simulink model "copy_inversed1"  (R2023b)
settings: Solver=VariableStepAuto  StartTime=0.0  StopTime=100  RelTol=1e-3
libraries: simulink_extras x2, slpidlib x1
settings Model: Creator=macbook  LastModifiedBy=user

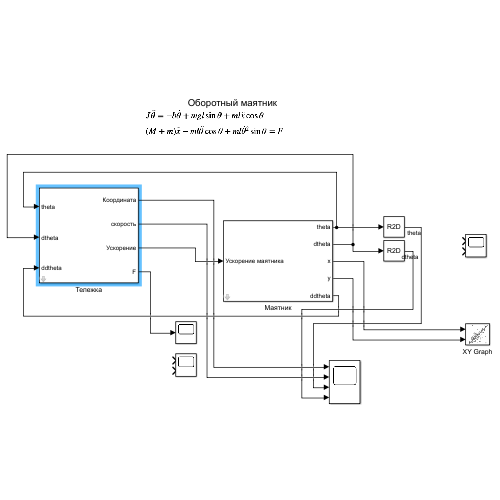
[thumbnail: Simulink's stored preview of the top-level diagram]
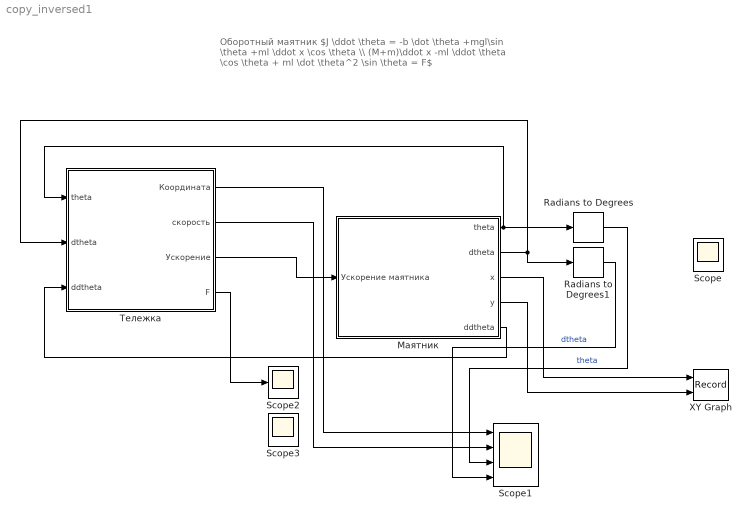
== system copy_inversed1 ==
  note: Оборотный маятник
      | $J \ddot \theta = -b \dot \theta +mgl\sin \theta +ml \ddot x \cos \theta \\ (M+m)\ddot x -ml \ddot \theta \cos \theta + ml \dot \theta^2 \sin \theta = F$
  Radians to Degrees : simulink_extras/Transformations/Radians to Degrees
  Radians to Degrees1 : simulink_extras/Transformations/Radians to Degrees
  Scope : Scope  NumInputPorts=2
  Scope1 : Scope  NumInputPorts=4
  Scope2 : Scope
  Scope3 : Scope  NumInputPorts=2
  XY Graph : Record  FileSettingsInternal="{\"entries\":[{\"content\":{\"excelSettings\":{\"content\":{},\"type\":\"Streamout.ExcelSettings\"}},\"type\":\"Streamout.FileSettingStorage\",\"uuid\":\"\"}],\"packageUris\":[\"http:\\/\\/schema.mathworks.com\\/mf0\\/streamout_blocks\\/R2020a\"],\"version\":\"1.0\"}"  Layout=[1 1]  SignalsInternal="{\"entries\":[{\"content\":{\"signals\":[{\"content\":{\"blockPath\":[],\"dimensions\":[1],\"domain\":\"\",\"lineColor\":\"#a2142f\",\"plots\":[1],\"port\":1,\"sid\":[\"\"],\"signalID\":125,\"signalName\":\"Маятник:3\"},\"type\":\"RecordBlkView.Signal\",\"uuid\":\"\"},{\"content\":{\"blockPath\":[],\"dimensions\":[1],\"domain\":\"\",\"lineColor\":\"#139fff\",\"plots\":[1],\"port\":2,\"sid\":[\"\"],\"signalID\":129,\"signalName\":\"Маятник:4\"},\"type\":\"RecordBlkView.Signal\",\"uuid\":\"\"}]},\"type\":\"RecordBlkView.InputSignals\",\"uuid\":\"\"}],\"packageUris\":[\"http:\\/\\/schema.mathworks.com\\/mf0\\/streamout_blocks\\/R2020a\"],\"version\":\"1.0\"}"  VisualizationBindings="{\"xyplotplugin\":{\"info\":[{\"series\":[{\"bindingParametersList\":[{\"parameter\":\"X-Axis\",\"signalID\":125,\"signalName\":\"Маятник:3\"},{\"parameter\":\"Y-Axis\",\"signalID\":129,\"signalName\":\"Маятник:4\"}],\"seriesID\":60754}],\"subplotID\":1}]}}"  CompatibilityTag=XY
  Маятник : Subsystem  mask{m=0.1, l=0.5, g=9.8, angel=20, b=0.05}
      mask prompts: angel "Начальный угол"
  Тележка : Subsystem  mask{F=0, Mas=1, m=0.1, l=0.5}
      mask prompts: F "начальная F"; Mas "M"
  wires:
  Маятник/1(theta) -> Тележка/1(theta), Radians to Degrees/1
  Radians to Degrees/1 -> Scope1/3  "theta"
  Маятник/3(x) -> XY Graph/1
  Маятник/2(dtheta) -> Тележка/2(dtheta), Radians to Degrees1/1
  Radians to Degrees1/1 -> Scope1/4  "dtheta"
  Маятник/4(y) -> XY Graph/2
  Тележка/4(F) -> Scope2/1
  Тележка/3(Ускорение) -> Маятник/1(Ускорение маятника)
  Маятник/5(ddtheta) -> Тележка/3(ddtheta)
  Тележка/1(Координата) -> Scope1/1
  Тележка/2(скорость) -> Scope1/2

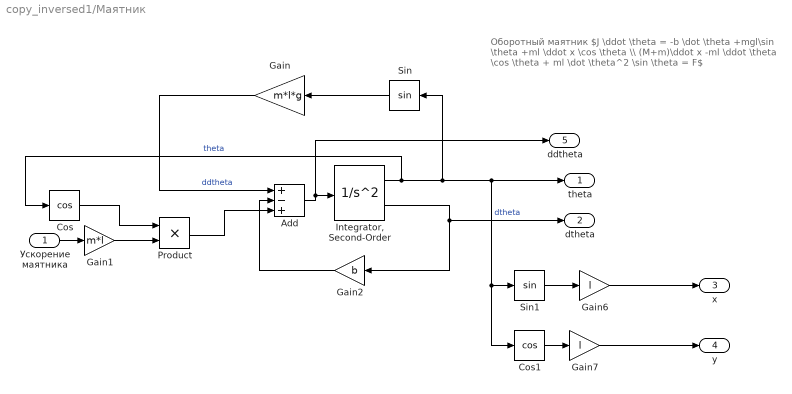
== system copy_inversed1/Маятник ==
  note: Оборотный маятник
      | $J \ddot \theta = -b \dot \theta +mgl\sin \theta +ml \ddot x \cos \theta \\ (M+m)\ddot x -ml \ddot \theta \cos \theta + ml \dot \theta^2 \sin \theta = F$
  Ускорение маятника : Inport
  Add : Sum  Inputs=+-+
  Cos : Trigonometry  Operator=cos
  Cos1 : Trigonometry  Operator=cos
  Gain : Gain  Gain=m*l*g
  Gain1 : Gain  Gain=m*l
  Gain2 : Gain  Gain=b
  Gain6 : Gain  Gain=l
  Gain7 : Gain  Gain=l
  "Integrator, Second-Order" : SecondOrderIntegrator  ICX=deg2rad(angel)  ICDXDT=0
  Product : Product
  Sin : Trigonometry
  Sin1 : Trigonometry
  theta : Outport
  dtheta : Outport  Port=2
  x : Outport  Port=3
  y : Outport  Port=4
  ddtheta : Outport  Port=5
  wires:
  Gain/1 -> Add/1  "ddtheta"
  Add/1 -> ddtheta/1, "Integrator, Second-Order"/1
  Sin1/1 -> Gain6/1
  Gain7/1 -> y/1
  Cos1/1 -> Gain7/1
  "Integrator, Second-Order"/2 -> Gain2/1, dtheta/1  "dtheta"
  "Integrator, Second-Order"/1 -> theta/1, Cos1/1, Sin1/1, Sin/1, Cos/1  "theta"
  Gain2/1 -> Add/2
  Gain6/1 -> x/1
  Sin/1 -> Gain/1
  Ускорение маятника/1 -> Gain1/1
  Gain1/1 -> Product/2
  Cos/1 -> Product/1
  Product/1 -> Add/3

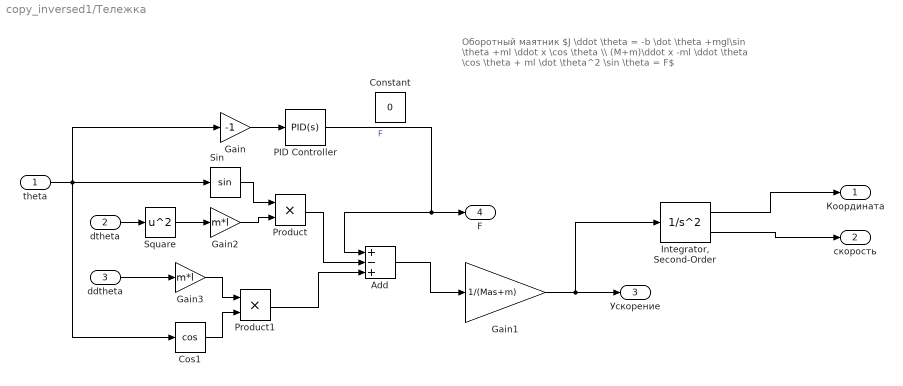
== system copy_inversed1/Тележка ==
  note: Оборотный маятник
      | $J \ddot \theta = -b \dot \theta +mgl\sin \theta +ml \ddot x \cos \theta \\ (M+m)\ddot x -ml \ddot \theta \cos \theta + ml \dot \theta^2 \sin \theta = F$
  theta : Inport
  dtheta : Inport  Port=2
  ddtheta : Inport  Port=3
  Add : Sum  Inputs=+-+
  Constant : Constant  Value=0
  Cos1 : Trigonometry  Operator=cos
  Gain : Gain  Gain=-1
  Gain1 : Gain  Gain=1/(Mas+m)
  Gain2 : Gain  Gain=m*l
  Gain3 : Gain  Gain=m*l
  "Integrator, Second-Order" : SecondOrderIntegrator
  PID Controller : slpidlib/PID Controller  Controller=PID  Form=Parallel  TimeDomain=Continuous-time  UseExternalTs=off  SampleTime=-1  IntegratorMethod=Forward Euler  FilterMethod=Forward Euler  ControllerParametersSource=internal  P=50  I=1  UseKiTs=on  D=50  N=100  UseFilter=on  TunerSelectOption=Transfer Function Based (PID Tuner App)  InitialConditionSource=internal  InitialConditionForIntegrator=0  InitialConditionForFilter=0  DifferentiatorICPrevScaledInput=0  ExternalReset=none  TrackingMode=off  Kt=1  LimitOutput=off  SatLimitsSource=internal  UpperSaturationLimit=inf  LowerSaturationLimit=-inf  LinearizeAsGain=on  AntiWindupMode=none  Kb=1  LimitIntegrator=off  UpperIntegratorSaturationLimit=inf  LowerIntegratorSaturationLimit=-inf  POutMin=[]  POutMax=[]  IOutMin=[]  IOutMax=[]  DOutMin=[]  DOutMax=[]  NOutMin=[]  NOutMax=[]  SumOutMin=[]  SumOutMax=[]  SaturationOutMin=[]  SaturationOutMax=[]  PParamMin=[]  PParamMax=[]  IParamMin=[]  IParamMax=[]  DParamMin=[]  DParamMax=[]  NParamMin=[]  NParamMax=[]  KbParamMin=[]  KbParamMax=[]  KtParamMin=[]  KtParamMax=[]  KbOutMin=[]  KbOutMax=[]  KtOutMin=[]  KtOutMax=[]  IntegratorOutMin=[]  IntegratorOutMax=[]  FilterOutMin=[]  FilterOutMax=[]  SumI1OutMin=[]  SumI1OutMax=[]  SumI2OutMin=[]  SumI2OutMax=[]  SumI3OutMin=[]  SumI3OutMax=[]  SumI4OutMin=[]  SumI4OutMax=[]  SumDOutMin=[]  SumDOutMax=[]  DifferentiatorOutMin=[]  DifferentiatorOutMax=[]  FilterDiffOutCoefMin=[]  FilterDiffOutCoefMax=[]  ReciprocalOutMin=[]  ReciprocalOutMax=[]  SumDenOutMin=[]  SumDenOutMax=[]  SumNumOutMin=[]  SumNumOutMax=[]  DivideOutMin=[]  DivideOutMax=[]  UdiffTsProdOutMin=[]  UdiffTsProdOutMax=[]  NTsProdOutMin=[]  NTsProdOutMax=[]  UintegralTsProdOutMin=[]  UintegralTsProdOutMax=[]  UngainTsProdOutMin=[]  UngainTsProdOutMax=[]  ClampingZeroOutDataTypeStr=Inherit: Inherit via back propagation  ClampingZeroOutMin=[]  ClampingZeroOutMax=[]  FilterDenConstantOutDataTypeStr=Inherit: Inherit via back propagation  FilterDenConstantOutMin=[]  FilterDenConstantOutMax=[]  PCopyOutDataTypeStr=Inherit: Inherit via back propagation  PCopyOutMin=[]  PCopyOutMax=[]  NCopyOutDataTypeStr=Inherit: Inherit via back propagation  NCopyOutMin=[]  NCopyOutMax=[]  IntegratorContinuousStateAttributes=''  IntegratorStateMustResolveToSignalObject=off  IntegratorRTWStateStorageClass=Auto  FilterContinuousStateAttributes=''  FilterStateMustResolveToSignalObject=off  FilterRTWStateStorageClass=Auto  ParallelPVariant=InternalParameters  IdealPVariant=Disabled  IVariant=InternalParameters  DVariant=InternalParameters  IntegratorVariant=Continuous  SatVariant=Disabled  AWVariant=Passthrough  PCopyVariant=Disabled  TRVariant=Disabled  FdbkBlocksVariant=Forward  IdealPFdbkVariant=Disabled  SatFdbkVariant=Disabled  DerivativeFilterVariant=ContFilter  NVariant=InternalParameters  NCopyVariant=Disabled  FilterICVariant=InternalICsFilter  IntegratorICVariant=InternalICs  ExternalResetVariant=Disabled  TRSumVariant=Passthrough  SumFdbkVariant=Disabled  SumVariant=Sum_PID  TsampFilterVariant=InternalTs  TsampNgainVariant=Passthrough  TsampIntegralVariant=Disabled_SignalSpec  ExternalSaturationOutDataTypeStr=Inherit: Same as second input
  Product : Product
  Product1 : Product
  Sin : Trigonometry
  Square : Math  Operator=square
  Координата : Outport
  скорость : Outport  Port=2
  Ускорение : Outport  Port=3
  F : Outport  Port=4
  wires:
  PID Controller/1 -> Add/1, F/1  "F"
  theta/1 -> Sin/1, Gain/1, Cos1/1
  Gain/1 -> PID Controller/1
  dtheta/1 -> Square/1
  Square/1 -> Gain2/1
  Sin/1 -> Product/1
  Gain2/1 -> Product/2
  ddtheta/1 -> Gain3/1
  Gain3/1 -> Product1/1
  Cos1/1 -> Product1/2
  Product/1 -> Add/2
  Product1/1 -> Add/3
  Add/1 -> Gain1/1
  Gain1/1 -> "Integrator, Second-Order"/1, Ускорение/1
  "Integrator, Second-Order"/1 -> Координата/1
  "Integrator, Second-Order"/2 -> скорость/1
